simulink model "Self_Model_3D"  (R2023b)
settings: Solver=VariableStepAuto  StartTime=0.0  StopTime=5  RelTol=1e-3
PostLoadFcn:
  | addpath(fileparts(get_param('Self_Model_3D','FileName')),'-begin'); init_lqr_model;
InitFcn:
  | init_lqr_model;
undefined symbols (not defined in the file or in its folder): lqr_model_config, X, Y, Z
libraries: sm_lib x61, nesl_utility x19, slpidlib x2
(part 1 of 3)
settings Model: Creator=Gary  LastModifiedBy=Gary

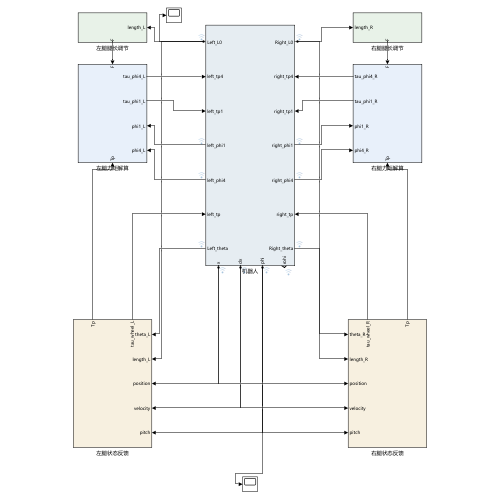
[thumbnail: Simulink's stored preview of the top-level diagram]
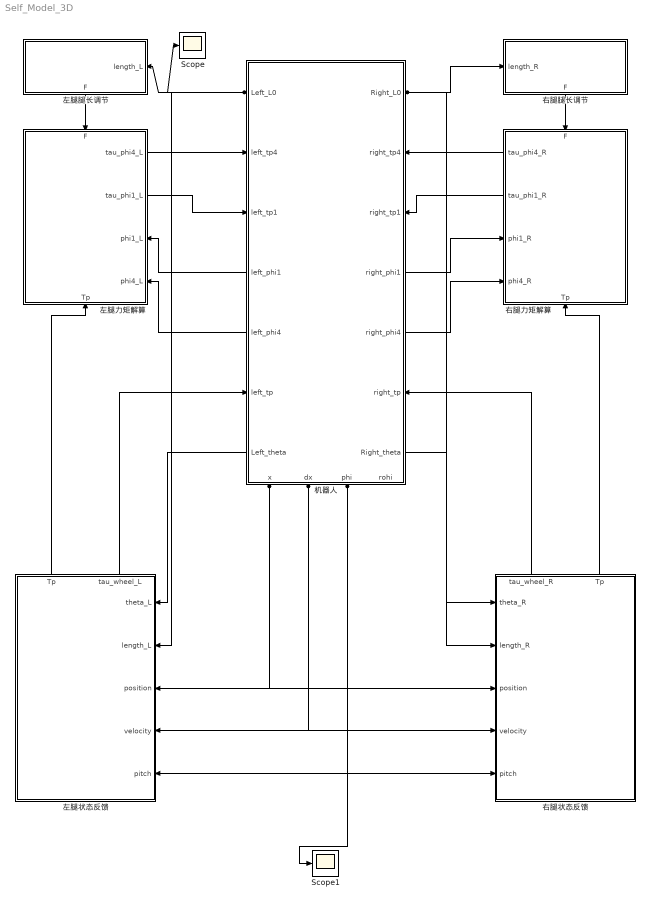
== system Self_Model_3D ==
  Scope : Scope
  Scope1 : Scope
  右腿力矩解算 : Subsystem
      settings: PortSchema="{\"entries\":[{\"content\":{\"sides\":[{\"content\":{\"connectorIds\":[\"Out1\",\"Out2\",\"In2\",\"In3\"],\"side\":\"LEFT\"},\"type\":\"ConnectorPlacement.EquallySpacedRectSide\",\"uuid\":\"cd193be0-05f5-4210-9b89-a5bff02ea1b3\"},{\"content\":{\"connectorIds\":[],\"side\":\"RIGHT\"},\"type\":\"ConnectorPlacement.EquallySpacedRectSide\",\"uuid\":\"1e2f5b89-c82e-4e0d-b2ce-74175c6e7738\"},{\"content\":{\"connectorIds\":[\"In1\"],\"side\":\"TOP\"},\"type\":\"ConnectorPlacement.EquallySpacedRectSide\",\"uuid\":\"9c87a6b9-8c47-4e9f-9491-dacb0d38e7db\"},{\"content\":{\"connectorIds\":[\"In4\"],\"side\":\"BOTTOM\"},\"type\":\"ConnectorPlacement.EquallySpacedRectSide\",\"uuid\":\"7c4cc001-f67c-4007-8028-1e7023a44da1\"}]},\"type\":\"ConnectorPlacement.EquallySpacedConnector\",\"uuid\":\"a103c52b-4f01-4ba1-8a51-8fe86b8d50f5\"}],\"packageUris\":[\"http://schema.mathworks.com/mf0/Connector/R2020b\"],\"version\":\"1.0\"}"
  右腿状态反馈 : Subsystem
      settings: PortSchema="{\"entries\":[{\"content\":{\"sides\":[{\"content\":{\"connectorIds\":[\"In3\",\"In4\",\"In2\",\"In1\",\"In5\"],\"side\":\"LEFT\"},\"type\":\"ConnectorPlacement.EquallySpacedRectSide\",\"uuid\":\"cd193be0-05f5-4210-9b89-a5bff02ea1b3\"},{\"content\":{\"connectorIds\":[],\"side\":\"RIGHT\"},\"type\":\"ConnectorPlacement.EquallySpacedRectSide\",\"uuid\":\"1e2f5b89-c82e-4e0d-b2ce-74175c6e7738\"},{\"content\":{\"connectorIds\":[\"Out2\",\"Out1\"],\"side\":\"TOP\"},\"type\":\"ConnectorPlacement.EquallySpacedRectSide\",\"uuid\":\"9c87a6b9-8c47-4e9f-9491-dacb0d38e7db\"},{\"content\":{\"connectorIds\":[],\"side\":\"BOTTOM\"},\"type\":\"ConnectorPlacement.EquallySpacedRectSide\",\"uuid\":\"7c4cc001-f67c-4007-8028-1e7023a44da1\"}]},\"type\":\"ConnectorPlacement.EquallySpacedConnector\",\"uuid\":\"a103c52b-4f01-4ba1-8a51-8fe86b8d50f5\"}],\"packageUris\":[\"http://schema.mathworks.com/mf0/Connector/R2020b\"],\"version\":\"1.0\"}"
  右腿腿长调节 : Subsystem
      settings: PortSchema="{\"entries\":[{\"content\":{\"sides\":[{\"content\":{\"connectorIds\":[\"In1\"],\"side\":\"LEFT\"},\"type\":\"ConnectorPlacement.EquallySpacedRectSide\",\"uuid\":\"cd193be0-05f5-4210-9b89-a5bff02ea1b3\"},{\"content\":{\"connectorIds\":[],\"side\":\"RIGHT\"},\"type\":\"ConnectorPlacement.EquallySpacedRectSide\",\"uuid\":\"1e2f5b89-c82e-4e0d-b2ce-74175c6e7738\"},{\"content\":{\"connectorIds\":[],\"side\":\"TOP\"},\"type\":\"ConnectorPlacement.EquallySpacedRectSide\",\"uuid\":\"9c87a6b9-8c47-4e9f-9491-dacb0d38e7db\"},{\"content\":{\"connectorIds\":[\"Out1\"],\"side\":\"BOTTOM\"},\"type\":\"ConnectorPlacement.EquallySpacedRectSide\",\"uuid\":\"7c4cc001-f67c-4007-8028-1e7023a44da1\"}]},\"type\":\"ConnectorPlacement.EquallySpacedConnector\",\"uuid\":\"a103c52b-4f01-4ba1-8a51-8fe86b8d50f5\"}],\"packageUris\":[\"http://schema.mathworks.com/mf0/Connector/R2020b\"],\"version\":\"1.0\"}"
  左腿力矩解算 : Subsystem
      settings: PortSchema="{\"entries\":[{\"content\":{\"sides\":[{\"content\":{\"connectorIds\":[],\"side\":\"LEFT\"},\"type\":\"ConnectorPlacement.EquallySpacedRectSide\",\"uuid\":\"cd193be0-05f5-4210-9b89-a5bff02ea1b3\"},{\"content\":{\"connectorIds\":[\"Out1\",\"Out2\",\"In2\",\"In3\"],\"side\":\"RIGHT\"},\"type\":\"ConnectorPlacement.EquallySpacedRectSide\",\"uuid\":\"1e2f5b89-c82e-4e0d-b2ce-74175c6e7738\"},{\"content\":{\"connectorIds\":[\"In1\"],\"side\":\"TOP\"},\"type\":\"ConnectorPlacement.EquallySpacedRectSide\",\"uuid\":\"9c87a6b9-8c47-4e9f-9491-dacb0d38e7db\"},{\"content\":{\"connectorIds\":[\"In4\"],\"side\":\"BOTTOM\"},\"type\":\"ConnectorPlacement.EquallySpacedRectSide\",\"uuid\":\"7c4cc001-f67c-4007-8028-1e7023a44da1\"}]},\"type\":\"ConnectorPlacement.EquallySpacedConnector\",\"uuid\":\"a103c52b-4f01-4ba1-8a51-8fe86b8d50f5\"}],\"packageUris\":[\"http://schema.mathworks.com/mf0/Connector/R2020b\"],\"version\":\"1.0\"}"
  左腿状态反馈 : Subsystem
      settings: PortSchema="{\"entries\":[{\"content\":{\"sides\":[{\"content\":{\"connectorIds\":[],\"side\":\"LEFT\"},\"type\":\"ConnectorPlacement.EquallySpacedRectSide\",\"uuid\":\"cd193be0-05f5-4210-9b89-a5bff02ea1b3\"},{\"content\":{\"connectorIds\":[\"In3\",\"In4\",\"In2\",\"In1\",\"In5\"],\"side\":\"RIGHT\"},\"type\":\"ConnectorPlacement.EquallySpacedRectSide\",\"uuid\":\"1e2f5b89-c82e-4e0d-b2ce-74175c6e7738\"},{\"content\":{\"connectorIds\":[\"Out1\",\"Out2\"],\"side\":\"TOP\"},\"type\":\"ConnectorPlacement.EquallySpacedRectSide\",\"uuid\":\"9c87a6b9-8c47-4e9f-9491-dacb0d38e7db\"},{\"content\":{\"connectorIds\":[],\"side\":\"BOTTOM\"},\"type\":\"ConnectorPlacement.EquallySpacedRectSide\",\"uuid\":\"7c4cc001-f67c-4007-8028-1e7023a44da1\"}]},\"type\":\"ConnectorPlacement.EquallySpacedConnector\",\"uuid\":\"a103c52b-4f01-4ba1-8a51-8fe86b8d50f5\"}],\"packageUris\":[\"http://schema.mathworks.com/mf0/Connector/R2020b\"],\"version\":\"1.0\"}"
  左腿腿长调节 : Subsystem
      settings: PortSchema="{\"entries\":[{\"content\":{\"sides\":[{\"content\":{\"connectorIds\":[],\"side\":\"LEFT\"},\"type\":\"ConnectorPlacement.EquallySpacedRectSide\",\"uuid\":\"cd193be0-05f5-4210-9b89-a5bff02ea1b3\"},{\"content\":{\"connectorIds\":[\"In1\"],\"side\":\"RIGHT\"},\"type\":\"ConnectorPlacement.EquallySpacedRectSide\",\"uuid\":\"1e2f5b89-c82e-4e0d-b2ce-74175c6e7738\"},{\"content\":{\"connectorIds\":[],\"side\":\"TOP\"},\"type\":\"ConnectorPlacement.EquallySpacedRectSide\",\"uuid\":\"9c87a6b9-8c47-4e9f-9491-dacb0d38e7db\"},{\"content\":{\"connectorIds\":[\"Out1\"],\"side\":\"BOTTOM\"},\"type\":\"ConnectorPlacement.EquallySpacedRectSide\",\"uuid\":\"7c4cc001-f67c-4007-8028-1e7023a44da1\"}]},\"type\":\"ConnectorPlacement.EquallySpacedConnector\",\"uuid\":\"a103c52b-4f01-4ba1-8a51-8fe86b8d50f5\"}],\"packageUris\":[\"http://schema.mathworks.com/mf0/Connector/R2020b\"],\"version\":\"1.0\"}"
  机器人 : Subsystem
      settings: PortSchema="{\"entries\":[{\"content\":{\"sides\":[{\"content\":{\"connectorIds\":[\"Out12\",\"In1\",\"In2\",\"Out10\",\"Out11\",\"In3\",\"Out9\"],\"side\":\"LEFT\"},\"type\":\"ConnectorPlacement.EquallySpacedRectSide\",\"uuid\":\"cd193be0-05f5-4210-9b89-a5bff02ea1b3\"},{\"content\":{\"connectorIds\":[\"Out4\",\"In4\",\"In5\",\"Out2\",\"Out3\",\"In6\",\"Out1\"],\"side\":\"RIGHT\"},\"type\":\"ConnectorPlacement.EquallySpacedRectSide\",\"uuid\":\"1e2f5b89-c82e-4e0d-b2ce-74175c6e7738\"},{\"content\":{\"connectorIds\":[],\"side\":\"TOP\"},\"type\":\"ConnectorPlacement.EquallySpacedRectSide\",\"uuid\":\"9c87a6b9-8c47-4e9f-9491-dacb0d38e7db\"},{\"content\":{\"connectorIds\":[\"Out7\",\"Out8\",\"Out5\",\"Out6\"],\"side\":\"BOTTOM\"},\"type\":\"ConnectorPlacement.EquallySpacedRectSide\",\"uuid\":\"7c4cc001-f67c-4007-8028-1e7023a44da1\"}]},\"type\":\"ConnectorPlacement.EquallySpacedConnector\",\"uuid\":\"a103c52b-4f01-4ba1-8a51-8fe86b8d50f5\"}],\"packageUris\":[\"http://schema.mathworks.com/mf0/Connector/R2020b\"],\"version\":\"1.0\"}"
  wires:
  右腿力矩解算/1(tau_phi4_R) -> 机器人/4(right_tp4)
  右腿力矩解算/2(tau_phi1_R) -> 机器人/5(right_tp1)
  右腿状态反馈/1(Tp) -> 右腿力矩解算/4(Tp)
  右腿状态反馈/2(tau_wheel_R) -> 机器人/6(right_tp)
  右腿腿长调节/1(F) -> 右腿力矩解算/1(F)
  左腿力矩解算/1(tau_phi4_L) -> 机器人/1(left_tp4)
  左腿力矩解算/2(tau_phi1_L) -> 机器人/2(left_tp1)
  左腿状态反馈/1(Tp) -> 左腿力矩解算/4(Tp)
  左腿状态反馈/2(tau_wheel_L) -> 机器人/3(left_tp)
  左腿腿长调节/1(F) -> 左腿力矩解算/1(F)
  机器人/1(Right_theta) -> 右腿状态反馈/3(theta_R)
  机器人/2(right_phi1) -> 右腿力矩解算/2(phi1_R)
  机器人/3(right_phi4) -> 右腿力矩解算/3(phi4_R)
  机器人/4(Right_L0) -> 右腿腿长调节/1(length_R), 右腿状态反馈/4(length_R)
  机器人/5(phi) -> 左腿状态反馈/5(pitch), 右腿状态反馈/5(pitch), Scope1/1
  机器人/7(x) -> 右腿状态反馈/2(position), 左腿状态反馈/2(position)
  机器人/8(dx) -> 右腿状态反馈/1(velocity), 左腿状态反馈/1(velocity)
  机器人/9(Left_theta) -> 左腿状态反馈/3(theta_L)
  机器人/10(left_phi1) -> 左腿力矩解算/2(phi1_L)
  机器人/11(left_phi4) -> 左腿力矩解算/3(phi4_L)
  机器人/12(Left_L0) -> 左腿状态反馈/4(length_L), Scope/1, 左腿腿长调节/1(length_L)

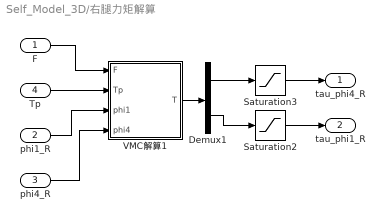
== system Self_Model_3D/右腿力矩解算 ==
  F : Inport
  phi1_R : Inport  Port=2
  phi4_R : Inport  Port=3
  Tp : Inport  Port=4
  Demux1 : Demux  Outputs=2
  Saturation2 : Saturate  UpperLimit=lqr_model_config.joint_torque_limit_nm  LowerLimit=-lqr_model_config.joint_torque_limit_nm  ZeroCross=off
  Saturation3 : Saturate  UpperLimit=lqr_model_config.joint_torque_limit_nm  LowerLimit=-lqr_model_config.joint_torque_limit_nm  ZeroCross=off
  VMC解算1 : MATLAB Function  TreatAsAtomicUnit=on
  tau_phi4_R : Outport
  tau_phi1_R : Outport  Port=2
  wires:
  Demux1/2 -> Saturation2/1
  phi4_R/1 -> VMC解算1/4(phi4)
  F/1 -> VMC解算1/1(F)
  Saturation3/1 -> tau_phi4_R/1
  phi1_R/1 -> VMC解算1/3(phi1)
  Tp/1 -> VMC解算1/2(Tp)
  VMC解算1/1(T) -> Demux1/1
  Demux1/1 -> Saturation3/1
  Saturation2/1 -> tau_phi1_R/1

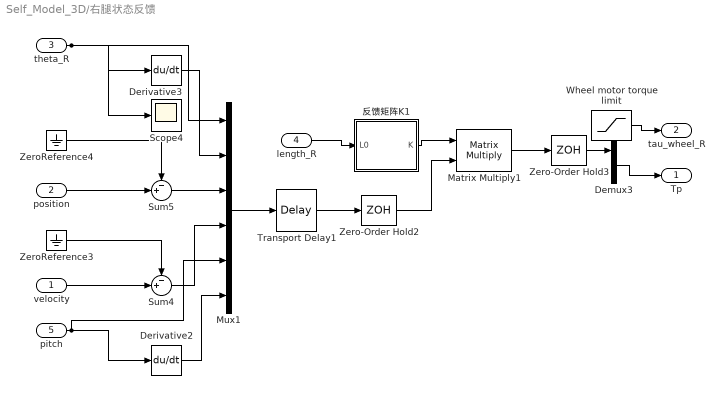
== system Self_Model_3D/右腿状态反馈 ==
  velocity : Inport
  position : Inport  Port=2
  theta_R : Inport  Port=3
  length_R : Inport  Port=4
  pitch : Inport  Port=5
  Demux3 : Demux  Outputs=2
  Derivative2 : Derivative
  Derivative3 : Derivative
  Matrix Multiply1 : Product  Multiplication=Matrix(*)
  Mux1 : Mux  Inputs=6
  Scope4 : Scope
  Sum4 : Sum  Inputs=-+|
  Sum5 : Sum  Inputs=-+|
  Transport Delay1 : TransportDelay  DelayTime=0
  Wheel motor torque limit : Saturate  UpperLimit=lqr_model_config.wheel_torque_limit_nm  LowerLimit=-lqr_model_config.wheel_torque_limit_nm  ZeroCross=off
  Zero-Order Hold2 : ZeroOrderHold  SampleTime=0.005
  Zero-Order Hold3 : ZeroOrderHold  SampleTime=0.005
  ZeroReference3 : Ground
  ZeroReference4 : Ground
  反馈矩阵K1 : MATLAB Function  TreatAsAtomicUnit=on
  Tp : Outport
  tau_wheel_R : Outport  Port=2
  wires:
  velocity/1 -> Sum4/2
  position/1 -> Sum5/2
  theta_R/1 -> Mux1/1, Derivative3/1, Scope4/1
  ZeroReference4/1 -> Sum5/1
  pitch/1 -> Mux1/5, Derivative2/1
  ZeroReference3/1 -> Sum4/1
  Derivative3/1 -> Mux1/2
  Sum5/1 -> Mux1/3
  Sum4/1 -> Mux1/4
  Derivative2/1 -> Mux1/6
  Mux1/1 -> Transport Delay1/1
  length_R/1 -> 反馈矩阵K1/1(L0)
  Transport Delay1/1 -> Zero-Order Hold2/1
  反馈矩阵K1/1(K) -> Matrix Multiply1/1
  Zero-Order Hold2/1 -> Matrix Multiply1/2
  Matrix Multiply1/1 -> Zero-Order Hold3/1
  Zero-Order Hold3/1 -> Demux3/1
  Demux3/2 -> Tp/1
  Demux3/1 -> Wheel motor torque limit/1
  Wheel motor torque limit/1 -> tau_wheel_R/1

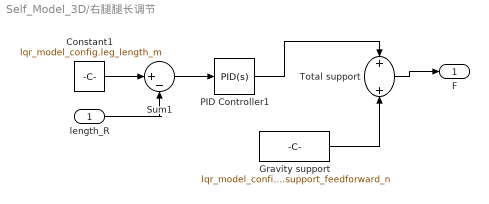
== system Self_Model_3D/右腿腿长调节 ==
  length_R : Inport
  Constant1 : Constant  Value=lqr_model_config.leg_length_m
  Gravity support : Constant  Value=lqr_model_config.support_feedforward_n
  PID Controller1 : slpidlib/PID Controller  Controller=PID  Form=Parallel  TimeDomain=Continuous-time  UseExternalTs=off  SampleTime=-1  IntegratorMethod=Forward Euler  FilterMethod=Forward Euler  ControllerParametersSource=internal  P=lqr_model_config.support_kp  I=lqr_model_config.support_ki  UseKiTs=off  D=lqr_model_config.support_kd  N=100  UseFilter=on  TunerSelectOption=Transfer Function Based (PID Tuner App)  InitialConditionSource=internal  InitialConditionForIntegrator=0  InitialConditionForFilter=0  DifferentiatorICPrevScaledInput=0  ExternalReset=none  TrackingMode=off  Kt=1  LimitOutput=off  SatLimitsSource=internal  UpperSaturationLimit=inf  LowerSaturationLimit=-inf  LinearizeAsGain=on  AntiWindupMode=none  Kb=1  LimitIntegrator=off  UpperIntegratorSaturationLimit=1.5  LowerIntegratorSaturationLimit=-1.5  POutMin=[]  POutMax=[]  IOutMin=[]  IOutMax=[]  DOutMin=[]  DOutMax=[]  NOutMin=[]  NOutMax=[]  SumOutMin=[]  SumOutMax=[]  SaturationOutMin=[]  SaturationOutMax=[]  PParamMin=[]  PParamMax=[]  IParamMin=[]  IParamMax=[]  DParamMin=[]  DParamMax=[]  NParamMin=[]  NParamMax=[]  KbParamMin=[]  KbParamMax=[]  KtParamMin=[]  KtParamMax=[]  KbOutMin=[]  KbOutMax=[]  KtOutMin=[]  KtOutMax=[]  IntegratorOutMin=[]  IntegratorOutMax=[]  FilterOutMin=[]  FilterOutMax=[]  SumI1OutMin=[]  SumI1OutMax=[]  SumI2OutMin=[]  SumI2OutMax=[]  SumI3OutMin=[]  SumI3OutMax=[]  SumI4OutMin=[]  SumI4OutMax=[]  SumDOutMin=[]  SumDOutMax=[]  DifferentiatorOutMin=[]  DifferentiatorOutMax=[]  FilterDiffOutCoefMin=[]  FilterDiffOutCoefMax=[]  ReciprocalOutMin=[]  ReciprocalOutMax=[]  SumDenOutMin=[]  SumDenOutMax=[]  SumNumOutMin=[]  SumNumOutMax=[]  DivideOutMin=[]  DivideOutMax=[]  UdiffTsProdOutMin=[]  UdiffTsProdOutMax=[]  NTsProdOutMin=[]  NTsProdOutMax=[]  UintegralTsProdOutMin=[]  UintegralTsProdOutMax=[]  UngainTsProdOutMin=[]  UngainTsProdOutMax=[]  ClampingZeroOutDataTypeStr=Inherit: Inherit via back propagation  ClampingZeroOutMin=[]  ClampingZeroOutMax=[]  FilterDenConstantOutDataTypeStr=Inherit: Inherit via back propagation  FilterDenConstantOutMin=[]  FilterDenConstantOutMax=[]  PCopyOutDataTypeStr=Inherit: Inherit via back propagation  PCopyOutMin=[]  PCopyOutMax=[]  NCopyOutDataTypeStr=Inherit: Inherit via back propagation  NCopyOutMin=[]  NCopyOutMax=[]  IntegratorContinuousStateAttributes=''  IntegratorStateMustResolveToSignalObject=off  IntegratorRTWStateStorageClass=Auto  FilterContinuousStateAttributes=''  FilterStateMustResolveToSignalObject=off  FilterRTWStateStorageClass=Auto  ParallelPVariant=InternalParameters  IdealPVariant=Disabled  IVariant=InternalParameters  DVariant=InternalParameters  IntegratorVariant=Continuous  SatVariant=Disabled  AWVariant=Passthrough  PCopyVariant=Disabled  TRVariant=Disabled  FdbkBlocksVariant=Forward  IdealPFdbkVariant=Disabled  SatFdbkVariant=Disabled  DerivativeFilterVariant=ContFilter  NVariant=InternalParameters  NCopyVariant=Disabled  FilterICVariant=InternalICsFilter  IntegratorICVariant=InternalICs  ExternalResetVariant=Disabled  TRSumVariant=Passthrough  SumFdbkVariant=Disabled  SumVariant=Sum_PID  TsampFilterVariant=InternalTs  TsampNgainVariant=Passthrough  TsampIntegralVariant=Disabled_SignalSpec  ExternalSaturationOutDataTypeStr=Inherit: Same as second input
  Sum1 : Sum  Inputs=|+-
  Total support : Sum
  F : Outport
  wires:
  Constant1/1 -> Sum1/1
  Sum1/1 -> PID Controller1/1
  length_R/1 -> Sum1/2
  PID Controller1/1 -> Total support/1
  Gravity support/1 -> Total support/2
  Total support/1 -> F/1

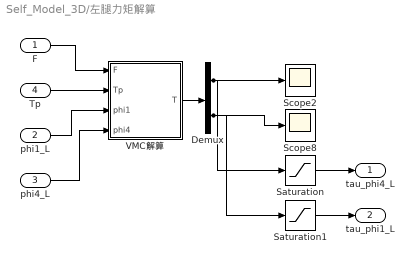
== system Self_Model_3D/左腿力矩解算 ==
  F : Inport
  phi1_L : Inport  Port=2
  phi4_L : Inport  Port=3
  Tp : Inport  Port=4
  Demux : Demux  Outputs=2
  Saturation : Saturate  UpperLimit=lqr_model_config.joint_torque_limit_nm  LowerLimit=-lqr_model_config.joint_torque_limit_nm  ZeroCross=off
  Saturation1 : Saturate  UpperLimit=lqr_model_config.joint_torque_limit_nm  LowerLimit=-lqr_model_config.joint_torque_limit_nm  ZeroCross=off
  Scope2 : Scope
  Scope8 : Scope
  VMC解算 : MATLAB Function  TreatAsAtomicUnit=on
  tau_phi4_L : Outport
  tau_phi1_L : Outport  Port=2
  wires:
  F/1 -> VMC解算/1(F)
  Tp/1 -> VMC解算/2(Tp)
  phi4_L/1 -> VMC解算/4(phi4)
  phi1_L/1 -> VMC解算/3(phi1)
  VMC解算/1(T) -> Demux/1
  Demux/1 -> Scope2/1, Saturation/1
  Saturation/1 -> tau_phi4_L/1
  Demux/2 -> Scope8/1, Saturation1/1
  Saturation1/1 -> tau_phi1_L/1

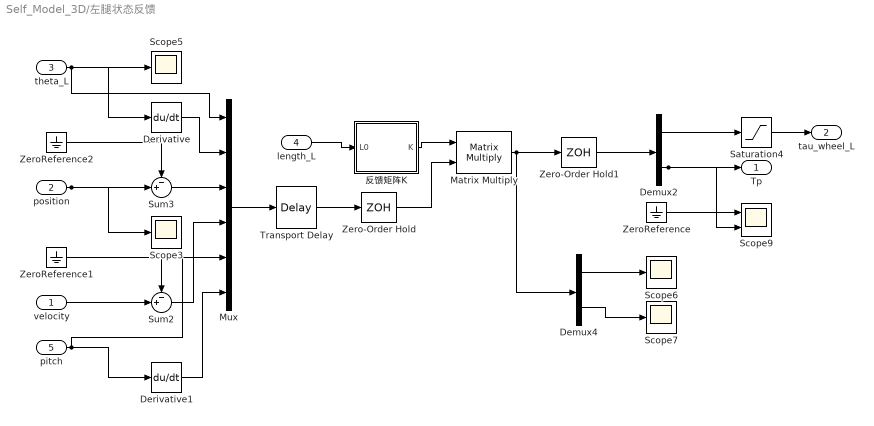
== system Self_Model_3D/左腿状态反馈 ==
  velocity : Inport
  position : Inport  Port=2
  theta_L : Inport  Port=3
  length_L : Inport  Port=4
  pitch : Inport  Port=5
  Demux2 : Demux  Outputs=2
  Demux4 : Demux  Outputs=2
  Derivative : Derivative
  Derivative1 : Derivative
  Matrix Multiply : Product  Multiplication=Matrix(*)
  Mux : Mux  Inputs=6
  Saturation4 : Saturate  UpperLimit=lqr_model_config.wheel_torque_limit_nm  LowerLimit=-lqr_model_config.wheel_torque_limit_nm  ZeroCross=off
  Scope{3,5..7} (4 alike) : Scope
  Scope9 : Scope  NumInputPorts=2
  Sum2 : Sum  Inputs=-+|
  Sum3 : Sum  Inputs=-+|
  Transport Delay : TransportDelay  DelayTime=0
  Zero-Order Hold : ZeroOrderHold  SampleTime=0.005
  Zero-Order Hold1 : ZeroOrderHold  SampleTime=0.005
  ZeroReference : Ground
  ZeroReference1 : Ground
  ZeroReference2 : Ground
  反馈矩阵K : MATLAB Function  TreatAsAtomicUnit=on
  Tp : Outport
  tau_wheel_L : Outport  Port=2
  wires:
  ZeroReference2/1 -> Sum3/1
  ZeroReference1/1 -> Sum2/1
  theta_L/1 -> Mux/1, Scope5/1, Derivative/1
  pitch/1 -> Derivative1/1, Mux/5
  position/1 -> Sum3/2, Scope3/1
  velocity/1 -> Sum2/2
  Derivative/1 -> Mux/2
  Sum3/1 -> Mux/3
  Sum2/1 -> Mux/4
  Derivative1/1 -> Mux/6
  Mux/1 -> Transport Delay/1
  length_L/1 -> 反馈矩阵K/1(L0)
  Transport Delay/1 -> Zero-Order Hold/1
  反馈矩阵K/1(K) -> Matrix Multiply/1
  Zero-Order Hold/1 -> Matrix Multiply/2
  Matrix Multiply/1 -> Demux4/1, Zero-Order Hold1/1
  Zero-Order Hold1/1 -> Demux2/1
  Demux4/1 -> Scope6/1
  Demux4/2 -> Scope7/1
  Demux2/1 -> Saturation4/1
  Demux2/2 -> Tp/1, Scope9/2
  ZeroReference/1 -> Scope9/1
  Saturation4/1 -> tau_wheel_L/1

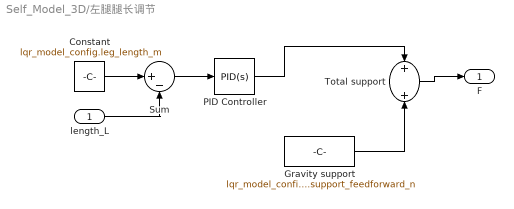
== system Self_Model_3D/左腿腿长调节 ==
  length_L : Inport
  Constant : Constant  Value=lqr_model_config.leg_length_m
  Gravity support : Constant  Value=lqr_model_config.support_feedforward_n
  PID Controller : slpidlib/PID Controller  Controller=PID  Form=Parallel  TimeDomain=Continuous-time  UseExternalTs=off  SampleTime=-1  IntegratorMethod=Forward Euler  FilterMethod=Forward Euler  ControllerParametersSource=internal  P=lqr_model_config.support_kp  I=lqr_model_config.support_ki  UseKiTs=off  D=lqr_model_config.support_kd  N=100  UseFilter=on  TunerSelectOption=Transfer Function Based (PID Tuner App)  InitialConditionSource=internal  InitialConditionForIntegrator=0  InitialConditionForFilter=0  DifferentiatorICPrevScaledInput=0  ExternalReset=none  TrackingMode=off  Kt=1  LimitOutput=off  SatLimitsSource=internal  UpperSaturationLimit=inf  LowerSaturationLimit=-inf  LinearizeAsGain=on  AntiWindupMode=none  Kb=1  LimitIntegrator=off  UpperIntegratorSaturationLimit=1.5  LowerIntegratorSaturationLimit=-1.5  POutMin=[]  POutMax=[]  IOutMin=[]  IOutMax=[]  DOutMin=[]  DOutMax=[]  NOutMin=[]  NOutMax=[]  SumOutMin=[]  SumOutMax=[]  SaturationOutMin=[]  SaturationOutMax=[]  PParamMin=[]  PParamMax=[]  IParamMin=[]  IParamMax=[]  DParamMin=[]  DParamMax=[]  NParamMin=[]  NParamMax=[]  KbParamMin=[]  KbParamMax=[]  KtParamMin=[]  KtParamMax=[]  KbOutMin=[]  KbOutMax=[]  KtOutMin=[]  KtOutMax=[]  IntegratorOutMin=[]  IntegratorOutMax=[]  FilterOutMin=[]  FilterOutMax=[]  SumI1OutMin=[]  SumI1OutMax=[]  SumI2OutMin=[]  SumI2OutMax=[]  SumI3OutMin=[]  SumI3OutMax=[]  SumI4OutMin=[]  SumI4OutMax=[]  SumDOutMin=[]  SumDOutMax=[]  DifferentiatorOutMin=[]  DifferentiatorOutMax=[]  FilterDiffOutCoefMin=[]  FilterDiffOutCoefMax=[]  ReciprocalOutMin=[]  ReciprocalOutMax=[]  SumDenOutMin=[]  SumDenOutMax=[]  SumNumOutMin=[]  SumNumOutMax=[]  DivideOutMin=[]  DivideOutMax=[]  UdiffTsProdOutMin=[]  UdiffTsProdOutMax=[]  NTsProdOutMin=[]  NTsProdOutMax=[]  UintegralTsProdOutMin=[]  UintegralTsProdOutMax=[]  UngainTsProdOutMin=[]  UngainTsProdOutMax=[]  ClampingZeroOutDataTypeStr=Inherit: Inherit via back propagation  ClampingZeroOutMin=[]  ClampingZeroOutMax=[]  FilterDenConstantOutDataTypeStr=Inherit: Inherit via back propagation  FilterDenConstantOutMin=[]  FilterDenConstantOutMax=[]  PCopyOutDataTypeStr=Inherit: Inherit via back propagation  PCopyOutMin=[]  PCopyOutMax=[]  NCopyOutDataTypeStr=Inherit: Inherit via back propagation  NCopyOutMin=[]  NCopyOutMax=[]  IntegratorContinuousStateAttributes=''  IntegratorStateMustResolveToSignalObject=off  IntegratorRTWStateStorageClass=Auto  FilterContinuousStateAttributes=''  FilterStateMustResolveToSignalObject=off  FilterRTWStateStorageClass=Auto  ParallelPVariant=InternalParameters  IdealPVariant=Disabled  IVariant=InternalParameters  DVariant=InternalParameters  IntegratorVariant=Continuous  SatVariant=Disabled  AWVariant=Passthrough  PCopyVariant=Disabled  TRVariant=Disabled  FdbkBlocksVariant=Forward  IdealPFdbkVariant=Disabled  SatFdbkVariant=Disabled  DerivativeFilterVariant=ContFilter  NVariant=InternalParameters  NCopyVariant=Disabled  FilterICVariant=InternalICsFilter  IntegratorICVariant=InternalICs  ExternalResetVariant=Disabled  TRSumVariant=Passthrough  SumFdbkVariant=Disabled  SumVariant=Sum_PID  TsampFilterVariant=InternalTs  TsampNgainVariant=Passthrough  TsampIntegralVariant=Disabled_SignalSpec  ExternalSaturationOutDataTypeStr=Inherit: Same as second input
  Sum : Sum  Inputs=|+-
  Total support : Sum
  F : Outport
  wires:
  length_L/1 -> Sum/2
  Constant/1 -> Sum/1
  Sum/1 -> PID Controller/1
  PID Controller/1 -> Total support/1
  Gravity support/1 -> Total support/2
  Total support/1 -> F/1

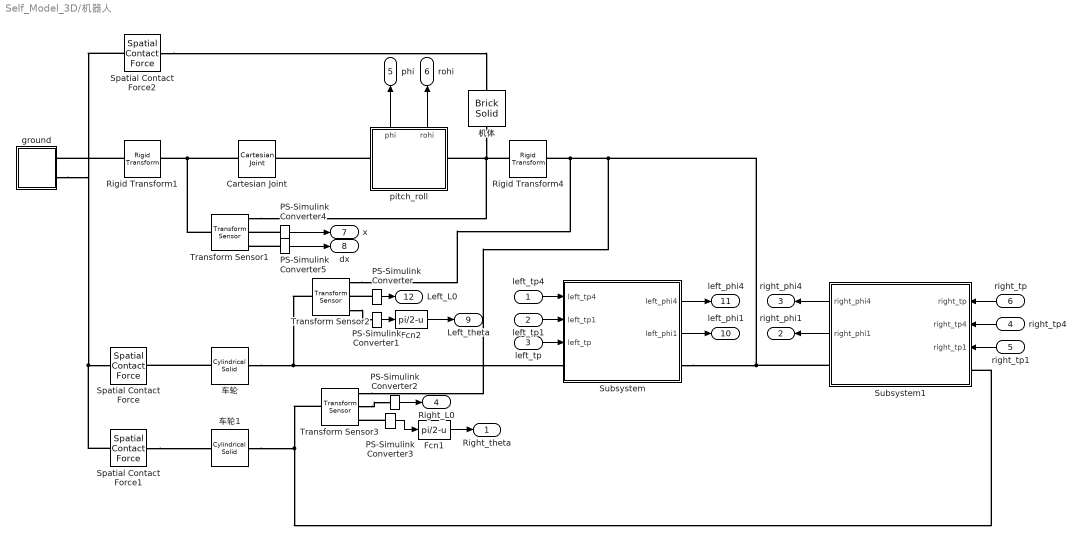
== system Self_Model_3D/机器人 ==
  left_tp4 : Inport
  left_tp1 : Inport  Port=2
  left_tp : Inport  Port=3
  right_tp4 : Inport  Port=4
  right_tp1 : Inport  Port=5
  right_tp : Inport  Port=6
  Cartesian Joint : sm_lib/Joints/Cartesian Joint  JointMode=Normal  SenseConstraintForce=off  SenseConstraintForceX=off  SenseConstraintForceY=off  SenseConstraintForceZ=off  SenseConstraintTorque=off  SenseConstraintTorqueX=off  SenseConstraintTorqueY=off  SenseConstraintTorqueZ=off  SenseTotalForce=off  SenseTotalForceX=off  SenseTotalForceY=off  SenseTotalForceZ=off  SenseTotalTorque=off  SenseTotalTorqueX=off  SenseTotalTorqueY=off  SenseTotalTorqueZ=off  CompositeWrenchDir=FollowerOnBase  CompositeWrenchFrame=BaseFrame  PxEquilibriumPosition=0  PxEquilibriumPositionUnits=m  PxSpringStiffness=0  PxSpringStiffnessUnits=N/m  PxDampingCoefficient=0  PxDampingCoefficientUnits=N/(m/s)  PxTorqueActuationMode=NoTorque  PxMotionActuationMode=ComputedMotion  PxSensePosition=off  PxSenseVelocity=off  PxSenseAcceleration=off  PxSenseTorqueForce=off  PxSenseLowerLimitTorqueForce=off  PxSenseUpperLimitTorqueForce=off  PxLowerLimitSpecify=off  PxLowerLimitBound=-1  PxLowerLimitBoundUnits=m  PxLowerLimitStiffness=1e6  PxLowerLimitStiffnessUnits=N/m  PxLowerLimitDamping=1e3  PxLowerLimitDampingUnits=N/(m/s)  PxLowerLimitTransitionRegionWidth=1e-4  PxLowerLimitTransitionRegionWidthUnits=m  PxUpperLimitSpecify=off  PxUpperLimitBound=1  PxUpperLimitBoundUnits=m  PxUpperLimitStiffness=1e6  PxUpperLimitStiffnessUnits=N/m  PxUpperLimitDamping=1e3  PxUpperLimitDampingUnits=N/(m/s)  PxUpperLimitTransitionRegionWidth=1e-4  PxUpperLimitTransitionRegionWidthUnits=m  PxPositionTargetSpecify=off  PxPositionTargetPriority=High  PxPositionTargetValue=0  PxPositionTargetValueUnits=m  PxVelocityTargetSpecify=off  PxVelocityTargetPriority=High  PxVelocityTargetValue=0  PxVelocityTargetValueUnits=m/s  PyEquilibriumPosition=0  PyEquilibriumPositionUnits=m  PySpringStiffness=0  PySpringStiffnessUnits=N/m  PyDampingCoefficient=0  PyDampingCoefficientUnits=N/(m/s)  PyTorqueActuationMode=NoTorque  PyMotionActuationMode=ComputedMotion  PySensePosition=off  PySenseVelocity=off  PySenseAcceleration=off  PySenseTorqueForce=off  PySenseLowerLimitTorqueForce=off  PySenseUpperLimitTorqueForce=off  PyLowerLimitSpecify=off  PyLowerLimitBound=-1  PyLowerLimitBoundUnits=m  PyLowerLimitStiffness=1e6  PyLowerLimitStiffnessUnits=N/m  PyLowerLimitDamping=1e3  PyLowerLimitDampingUnits=N/(m/s)  PyLowerLimitTransitionRegionWidth=1e-4  PyLowerLimitTransitionRegionWidthUnits=m  PyUpperLimitSpecify=off  PyUpperLimitBound=1  PyUpperLimitBoundUnits=m  PyUpperLimitStiffness=1e6  PyUpperLimitStiffnessUnits=N/m  PyUpperLimitDamping=1e3  PyUpperLimitDampingUnits=N/(m/s)  PyUpperLimitTransitionRegionWidth=1e-4  PyUpperLimitTransitionRegionWidthUnits=m  PyPositionTargetSpecify=off  PyPositionTargetPriority=High  PyPositionTargetValue=0  PyPositionTargetValueUnits=m  PyVelocityTargetSpecify=off  PyVelocityTargetPriority=High  PyVelocityTargetValue=0  PyVelocityTargetValueUnits=m/s  PzEquilibriumPosition=0  PzEquilibriumPositionUnits=m  PzSpringStiffness=0  PzSpringStiffnessUnits=N/m  PzDampingCoefficient=0  PzDampingCoefficientUnits=N/(m/s)  PzTorqueActuationMode=NoTorque  PzMotionActuationMode=ComputedMotion  PzSensePosition=off  PzSenseVelocity=off  PzSenseAcceleration=off  PzSenseTorqueForce=off  PzSenseLowerLimitTorqueForce=off  PzSenseUpperLimitTorqueForce=off  PzLowerLimitSpecify=off  PzLowerLimitBound=-1  PzLowerLimitBoundUnits=m  PzLowerLimitStiffness=1e6  PzLowerLimitStiffnessUnits=N/m  PzLowerLimitDamping=1e3  PzLowerLimitDampingUnits=N/(m/s)  PzLowerLimitTransitionRegionWidth=1e-4  PzLowerLimitTransitionRegionWidthUnits=m  PzUpperLimitSpecify=off  PzUpperLimitBound=1  PzUpperLimitBoundUnits=m  PzUpperLimitStiffness=1e6  PzUpperLimitStiffnessUnits=N/m  PzUpperLimitDamping=1e3  PzUpperLimitDampingUnits=N/(m/s)  PzUpperLimitTransitionRegionWidth=1e-4  PzUpperLimitTransitionRegionWidthUnits=m  PzPositionTargetSpecify=off  PzPositionTargetPriority=High  PzPositionTargetValue=0  PzPositionTargetValueUnits=m  PzVelocityTargetSpecify=off  PzVelocityTargetPriority=High  PzVelocityTargetValue=0  PzVelocityTargetValueUnits=m/s
  Fcn1 : Fcn  Expr=pi/2-u
  Fcn2 : Fcn  Expr=pi/2-u
  PS-Simulink Converter{,1..5} (6 alike) : nesl_utility/PS-Simulink Converter  PhysicalDomain=network_engine_domain  SubClassName=ps_output  LeftPortType=input  RightPortType=output  PseudoPeriodic=off  Frequencies=[]  VectorFormat=inherit  Unit=inherit  AffineConversion=off
  Rigid Transform1 : sm_lib/Frames and Transforms/Rigid Transform  TranslationMethod=StandardAxis  TranslationStandardOffset=lqr_model_config.body_initial_height_m  TranslationStandardOffsetUnits=m  TranslationStandardAxis=+Y  TranslationCartesianOffset=[0 0 0]  TranslationCartesianOffsetUnits=m  TranslationROffset=0  TranslationROffsetUnits=m  TranslationZOffset=0  TranslationZOffsetUnits=m  TranslationThetaOffset=0  TranslationThetaOffsetUnits=deg  RotationMethod=None  RotationAngleUnits=deg  RotationStandardAxis=+Z  RotationAngle=0.0  RotationArbitraryAxis=[0 0 1]  FollAlignAxisA=+X  BaseAlignAxisA=+Y  FollAlignAxisB=+Y  BaseAlignAxisB=+Z  RotationSequenceAxes=FollowerAxes  RotationSequence=XYX  RotationSequenceAngles=[0 0 0]  RotationSequenceAnglesUnits=deg  RotationMatrix=[1 0 0; 0 1 0; 0 0 1]  Quaternion=[1 0 0 0]
  Rigid Transform4 : sm_lib/Frames and Transforms/Rigid Transform  TranslationMethod=StandardAxis  TranslationStandardOffset=0.01  TranslationStandardOffsetUnits=m  TranslationStandardAxis=-Y  TranslationCartesianOffset=[0 0 0]  TranslationCartesianOffsetUnits=m  TranslationROffset=0  TranslationROffsetUnits=m  TranslationZOffset=0  TranslationZOffsetUnits=m  TranslationThetaOffset=0  TranslationThetaOffsetUnits=deg  RotationMethod=None  RotationAngleUnits=deg  RotationStandardAxis=+Z  RotationAngle=0.0  RotationArbitraryAxis=[0 0 1]  FollAlignAxisA=+X  BaseAlignAxisA=+Y  FollAlignAxisB=+Y  BaseAlignAxisB=+Z  RotationSequenceAxes=FollowerAxes  RotationSequence=XYX  RotationSequenceAngles=[0 0 0]  RotationSequenceAnglesUnits=deg  RotationMatrix=[1 0 0; 0 1 0; 0 0 1]  Quaternion=[1 0 0 0]
  Spatial Contact Force : sm_lib/Forces and Torques/Spatial Contact Force  SenseContactBaseRotation=off  SenseContactBaseTranslation=off  CoefficientOfDynamicFriction=0.3  CoefficientOfStaticFriction=0.5  NormalDamping=1e3  NormalDampingUnits=N/(m/s)  SenseContactSignal=off  NormalStiffness=1e6  NormalStiffnessUnits=N/m  FrictionalCriticalVelocity=1e-3  FrictionalCriticalVelocityUnits=m/s  ZeroCrossDetectContactStartAndEnd=off  SenseContactFollowerRotation=off  SenseContactFollowerTranslation=off  FrictionType=SmoothStickSlip  SenseFrictionalForceMagnitude=off  SenseNormalForceMagnitude=off  NormalForceType=SmoothSpringDamper  SenseNormalVelocity=off  SensePenetrationDepth=off  SenseSeparationDistance=off  SenseTangentialVelocity=off  NormalTransitionRegionWidth=1e-4  NormalTransitionRegionWidthUnits=m
  Spatial Contact Force1 : sm_lib/Forces and Torques/Spatial Contact Force  SenseContactBaseRotation=off  SenseContactBaseTranslation=off  CoefficientOfDynamicFriction=0.3  CoefficientOfStaticFriction=0.5  NormalDamping=1e3  NormalDampingUnits=N/(m/s)  SenseContactSignal=off  NormalStiffness=1e6  NormalStiffnessUnits=N/m  FrictionalCriticalVelocity=1e-3  FrictionalCriticalVelocityUnits=m/s  ZeroCrossDetectContactStartAndEnd=off  SenseContactFollowerRotation=off  SenseContactFollowerTranslation=off  FrictionType=SmoothStickSlip  SenseFrictionalForceMagnitude=off  SenseNormalForceMagnitude=off  NormalForceType=SmoothSpringDamper  SenseNormalVelocity=off  SensePenetrationDepth=off  SenseSeparationDistance=off  SenseTangentialVelocity=off  NormalTransitionRegionWidth=1e-4  NormalTransitionRegionWidthUnits=m
  Spatial Contact Force2 : sm_lib/Forces and Torques/Spatial Contact Force  SenseContactBaseRotation=off  SenseContactBaseTranslation=off  CoefficientOfDynamicFriction=0.3  CoefficientOfStaticFriction=0.5  NormalDamping=1e3  NormalDampingUnits=N/(m/s)  SenseContactSignal=off  NormalStiffness=1e6  NormalStiffnessUnits=N/m  FrictionalCriticalVelocity=1e-3  FrictionalCriticalVelocityUnits=m/s  ZeroCrossDetectContactStartAndEnd=off  SenseContactFollowerRotation=off  SenseContactFollowerTranslation=off  FrictionType=SmoothStickSlip  SenseFrictionalForceMagnitude=off  SenseNormalForceMagnitude=off  NormalForceType=SmoothSpringDamper  SenseNormalVelocity=off  SensePenetrationDepth=off  SenseSeparationDistance=off  SenseTangentialVelocity=off  NormalTransitionRegionWidth=1e-4  NormalTransitionRegionWidthUnits=m
  Subsystem : Subsystem
  Subsystem1 : Subsystem
      settings: PortSchema="{\"entries\":[{\"content\":{\"sides\":[{\"content\":{\"connectorIds\":[\"Out1\",\"Out2\",\"LConn1\"]},\"type\":\"ConnectorPlacement.EquallySpacedRectSide\",\"uuid\":\"8bfabdab-878d-48c0-a11e-de3a6c0ab8b0\"},{\"content\":{\"connectorIds\":[\"In1\",\"In2\",\"In3\",\"RConn1\"],\"side\":\"RIGHT\"},\"type\":\"ConnectorPlacement.EquallySpacedRectSide\",\"uuid\":\"ccc39fe7-f22e-4523-845a-484f8e0dd2bc\"},{\"content\":{\"side\":\"TOP\"},\"type\":\"ConnectorPlacement.EquallySpacedRectSide\",\"uuid\":\"206048fa-15f1-4370-a3cf-56c49d445876\"}]},\"type\":\"ConnectorPlacement.EquallySpacedConnector\",\"uuid\":\"c99860b8-29ef-46cc-9207-484f815784d8\"}],\"packageUris\":[\"http://schema.mathworks.com/mf0/Connector/R2020b\"],\"version\":\"1.0\"}"
  Transform Sensor1 : sm_lib/Frames and Transforms/Transform Sensor  MeasurementFrame=World  RotationSequence=XYX  SenseAngle=off  SenseAxis=off  SenseQ=off  SenseR=off  SenseRotationSequence=off  SenseOmegaX=off  SenseOmegaY=off  SenseOmegaZ=off  SenseOmega=off  SenseQDot=off  SenseRDot=off  SenseRotationSequenceDot=off  SenseAlphaX=off  SenseAlphaY=off  SenseAlphaZ=off  SenseAlpha=off  SenseQDDot=off  SenseRDDot=off  SenseX=on  SenseY=off  SenseZ=off  SenseXYZ=off  SenseRad=off  SenseAzim=off  SenseDist=off  SenseInc=off  SenseXDot=on  SenseYDot=off  SenseZDot=off  SenseXYZDot=off  SenseRadDot=off  SenseAzimDot=off  SenseDistDot=off  SenseIncDot=off  SenseXDDot=off  SenseYDDot=off  SenseZDDot=off  SenseXYZDDot=off  SenseRadDDot=off  SenseAzimDDot=off  SenseDistDDot=off  SenseIncDDot=off
  Transform Sensor2 : sm_lib/Frames and Transforms/Transform Sensor  MeasurementFrame=World  RotationSequence=XYX  SenseAngle=off  SenseAxis=off  SenseQ=off  SenseR=off  SenseRotationSequence=off  SenseOmegaX=off  SenseOmegaY=off  SenseOmegaZ=off  SenseOmega=off  SenseQDot=off  SenseRDot=off  SenseRotationSequenceDot=off  SenseAlphaX=off  SenseAlphaY=off  SenseAlphaZ=off  SenseAlpha=off  SenseQDDot=off  SenseRDDot=off  SenseX=off  SenseY=off  SenseZ=off  SenseXYZ=off  SenseRad=on  SenseAzim=on  SenseDist=off  SenseInc=off  SenseXDot=off  SenseYDot=off  SenseZDot=off  SenseXYZDot=off  SenseRadDot=off  SenseAzimDot=off  SenseDistDot=off  SenseIncDot=off  SenseXDDot=off  SenseYDDot=off  SenseZDDot=off  SenseXYZDDot=off  SenseRadDDot=off  SenseAzimDDot=off  SenseDistDDot=off  SenseIncDDot=off
  Transform Sensor3 : sm_lib/Frames and Transforms/Transform Sensor  MeasurementFrame=World  RotationSequence=XYX  SenseAngle=off  SenseAxis=off  SenseQ=off  SenseR=off  SenseRotationSequence=off  SenseOmegaX=off  SenseOmegaY=off  SenseOmegaZ=off  SenseOmega=off  SenseQDot=off  SenseRDot=off  SenseRotationSequenceDot=off  SenseAlphaX=off  SenseAlphaY=off  SenseAlphaZ=off  SenseAlpha=off  SenseQDDot=off  SenseRDDot=off  SenseX=off  SenseY=off  SenseZ=off  SenseXYZ=off  SenseRad=on  SenseAzim=on  SenseDist=off  SenseInc=off  SenseXDot=off  SenseYDot=off  SenseZDot=off  SenseXYZDot=off  SenseRadDot=off  SenseAzimDot=off  SenseDistDot=off  SenseIncDot=off  SenseXDDot=off  SenseYDDot=off  SenseZDDot=off  SenseXYZDDot=off  SenseRadDDot=off  SenseAzimDDot=off  SenseDistDDot=off  SenseIncDDot=off
  ground : Subsystem
  pitch_roll : Subsystem
      settings: PortSchema="{\"entries\":[{\"content\":{\"sides\":[{\"content\":{\"connectorIds\":[\"LConn1\"]},\"type\":\"ConnectorPlacement.EquallySpacedRectSide\",\"uuid\":\"fef6f933-62d5-45e7-ac96-e8cbafb6528b\"},{\"content\":{\"connectorIds\":[\"RConn1\"],\"side\":\"RIGHT\"},\"type\":\"ConnectorPlacement.EquallySpacedRectSide\",\"uuid\":\"177f9c9e-4cea-4eeb-a749-51d1f40b5813\"},{\"content\":{\"connectorIds\":[\"Out1\",\"Out2\"],\"side\":\"TOP\"},\"type\":\"ConnectorPlacement.EquallySpacedRectSide\",\"uuid\":\"706fbb75-e0e8-4abd-86a8-826d2da25550\"}]},\"type\":\"ConnectorPlacement.EquallySpacedConnector\",\"uuid\":\"210cb716-874d-4a12-866f-a9b733490919\"}],\"packageUris\":[\"http://schema.mathworks.com/mf0/Connector/R2020b\"],\"version\":\"1.0\"}"
  机体 : sm_lib/Body Elements/Brick Solid  GraphicAmbientColor=[0.15 0.15 0.15 1.0]  BasedOnType=Mass  BrickDimensions=[lqr_model_config.body_length_m lqr_model_config.body_height_m lqr_model_config.body_width_m]  BrickDimensionsUnits=m  CenterOfMass=[0 0 0]  CenterOfMassUnits=m  GraphicDiffuseColor=[0.5 0.5 0.5]  Density=1300  DensityUnits=kg/m^3  DoExposeReferenceFrame=on  GraphicEmissiveColor=[0.0 0.0 0.0 1.0]  ExportEntireGeometry=on  SerializedFrames=<Frames/>  MarkerShape=Sphere  MarkerSize=10  GraphicType=FromGeometry  InertiaType=CalculateFromGeometry  Mass=lqr_model_config.body_mass_kg  MassUnits=kg  MomentsOfInertia=[1 1 1]  MomentsOfInertiaUnits=kg*m^2  GraphicOpacity=1.0  ProductsOfInertia=[0 0 0]  ProductsOfInertiaUnits=kg*m^2  GraphicShininess=75  GraphicSpecularColor=[0.5 0.5 0.5 1.0]  GraphicVisPropType=SimpleVisualProperties
  车轮 : sm_lib/Body Elements/Cylindrical Solid  GraphicAmbientColor=[0.15 0.15 0.15 1.0]  BasedOnType=Density  CenterOfMass=[0 0 0]  CenterOfMassUnits=m  GraphicDiffuseColor=[0.5 0.5 0.5]  CylinderLength=lqr_model_config.wheel_width_m  CylinderLengthUnits=m  CylinderRadius=lqr_model_config.wheel_radius_m  CylinderRadiusUnits=m  Density=lqr_model_config.wheel_density_kg_m3  DensityUnits=kg/m^3  DoExposeReferenceFrame=on  GraphicEmissiveColor=[0.0 0.0 0.0 1.0]  ExportEntireGeometry=on  SerializedFrames=<Frames/>  MarkerShape=Sphere  MarkerSize=10  GraphicType=FromGeometry  InertiaType=CalculateFromGeometry  Mass=1  MassUnits=kg  MomentsOfInertia=[1 1 1]  MomentsOfInertiaUnits=kg*m^2  GraphicOpacity=1.0  ProductsOfInertia=[0 0 0]  ProductsOfInertiaUnits=kg*m^2  GraphicShininess=75  GraphicSpecularColor=[0.5 0.5 0.5 1.0]  GraphicVisPropType=SimpleVisualProperties
  车轮1 : sm_lib/Body Elements/Cylindrical Solid  GraphicAmbientColor=[0.15 0.15 0.15 1.0]  BasedOnType=Density  CenterOfMass=[0 0 0]  CenterOfMassUnits=m  GraphicDiffuseColor=[0.5 0.5 0.5]  CylinderLength=lqr_model_config.wheel_width_m  CylinderLengthUnits=m  CylinderRadius=lqr_model_config.wheel_radius_m  CylinderRadiusUnits=m  Density=lqr_model_config.wheel_density_kg_m3  DensityUnits=kg/m^3  DoExposeReferenceFrame=on  GraphicEmissiveColor=[0.0 0.0 0.0 1.0]  ExportEntireGeometry=on  SerializedFrames=<Frames/>  MarkerShape=Sphere  MarkerSize=10  GraphicType=FromGeometry  InertiaType=CalculateFromGeometry  Mass=1  MassUnits=kg  MomentsOfInertia=[1 1 1]  MomentsOfInertiaUnits=kg*m^2  GraphicOpacity=1.0  ProductsOfInertia=[0 0 0]  ProductsOfInertiaUnits=kg*m^2  GraphicShininess=75  GraphicSpecularColor=[0.5 0.5 0.5 1.0]  GraphicVisPropType=SimpleVisualProperties
  Right_theta : Outport
  right_phi1 : Outport  Port=2
  right_phi4 : Outport  Port=3
  Right_L0 : Outport  Port=4
  phi : Outport  Port=5
  rohi : Outport  Port=6
  x : Outport  Port=7
  dx : Outport  Port=8
  Left_theta : Outport  Port=9
  left_phi1 : Outport  Port=10
  left_phi4 : Outport  Port=11
  Left_L0 : Outport  Port=12
  wires:
  PS-Simulink Converter/1 -> Left_L0/1
  PS-Simulink Converter1/1 -> Fcn2/1
  Subsystem1/2(right_phi1) -> right_phi1/1
  PS-Simulink Converter2/1 -> Right_L0/1
  PS-Simulink Converter5/1 -> dx/1
  Subsystem1/1(right_phi4) -> right_phi4/1
  Fcn2/1 -> Left_theta/1
  PS-Simulink Converter4/1 -> x/1
  left_tp1/1 -> Subsystem/2(left_tp1)
  pitch_roll/2(rohi) -> rohi/1
  right_tp/1 -> Subsystem1/1(right_tp)
  pitch_roll/1(phi) -> phi/1
  right_tp4/1 -> Subsystem1/2(right_tp4)
  left_tp4/1 -> Subsystem/1(left_tp4)
  Subsystem/1(left_phi4) -> left_phi4/1
  Subsystem/2(left_phi1) -> left_phi1/1
  left_tp/1 -> Subsystem/3(left_tp)
  right_tp1/1 -> Subsystem1/3(right_tp1)
  PS-Simulink Converter3/1 -> Fcn1/1
  Fcn1/1 -> Right_theta/1
  connections:
  Subsystem/RConn1 -- Subsystem1/LConn1 -- Transform Sensor3/RConn1 -- Transform Sensor2/RConn1 -- Rigid Transform4/RConn1
  pitch_roll/LConn1 -- Cartesian Joint/RConn1
  车轮/RConn1 -- Transform Sensor2/LConn1 -- Subsystem/LConn1
  PS-Simulink Converter/LConn1 -- Transform Sensor2/RConn2
  Transform Sensor2/RConn3 -- PS-Simulink Converter1/LConn1
  车轮/LConn1 -- Spatial Contact Force/RConn1
  车轮1/RConn1 -- Transform Sensor3/LConn1 -- Subsystem1/RConn1
  PS-Simulink Converter4/LConn1 -- Transform Sensor1/RConn2
  PS-Simulink Converter5/LConn1 -- Transform Sensor1/RConn3
  Cartesian Joint/LConn1 -- Transform Sensor1/LConn1 -- Rigid Transform1/RConn1
  机体/RConn1 -- Transform Sensor1/RConn1 -- Rigid Transform4/LConn1 -- pitch_roll/RConn1
  Spatial Contact Force1/LConn1 -- Spatial Contact Force2/LConn1 -- ground/LConn2 -- Spatial Contact Force/LConn1
  Spatial Contact Force1/RConn1 -- 车轮1/LConn1
  Rigid Transform1/LConn1 -- ground/LConn1
  Spatial Contact Force2/RConn1 -- 机体/LConn1
  Transform Sensor3/RConn2 -- PS-Simulink Converter2/LConn1
  PS-Simulink Converter3/LConn1 -- Transform Sensor3/RConn3
